simulink model "IEEE13_coord"  (R2024b)
settings: Solver=ode4  StartTime=0.0  StopTime=1.3  FixedStep=Ts  MaxStep=1e-4  RelTol=1e-4
InitFcn:
  | a=1; % Loading Factor
  | Ts=50e-6;
  | % phase to sequence conversion of RXB matrices
  | c=1*exp(sqrt(-1)*(120*pi/180));
  | T=[1 1 1;1 c*c c;1 c c*c];
  | Tinv=1/3*[1 1 1;1 c c*c;1 c*c c];
  | 
  | % Simulation data for the IEEE 13 Node Test Feeder model
  | mi2km = 1.60934;%  miles to km conversion
  | ft2km = 0.0003048; % feet to km conversion
  | ms2F = 1*1e-6/(2*pi*60);% microsiemens to Farads conversion
  | 
  | 
  | %% Configuration 601
  | % Series Resitance and Reactance - ohm/mile
  | R_601 = [0.3465 0.1560 0.1580;0.1560 0.3375 0.1535;0.1580 0.1535 0.3414];
  | X_601 = [1.1079 0.5017 0.4236;0.5017 1.0478 0.3849;0.4236 0.3849 1.0348];
  | % charging susceptance - microsiemens/mile
  | B_601 = [6.2998 -1.9958 -1.2595;-1.9958 5.9597 -0.7417;-1.2595 -0.7417 5.6386];
  | 
  | R_601 = R_601/mi2km;
  | Rseq=Tinv*R_601*T;
  | R1_601=Rseq(2,2);R0_601=Rseq(1,1);
  | 
  | L_601 = (X_601/(2*pi*60))/mi2km;
  | Lseq=Tinv*L_601*T;
  | L1_601=Lseq(2,2);L0_601=Lseq(1,1);
  | 
  | C_601 =(B_601*ms2F)/mi2km;
  | Cseq=Tinv*C_601*T;
  | C1_601=Cseq(2,2);C0_601=Cseq(1,1);
  | 
  | %% Configuration 602 - series reactance - ohm/mile
  | R_602 = [0.7526 0.1580 0.1560;0.1580 0.7475 0.1535;0.1560 0.1535 0.7436];
  | X_602 = [1.1814 0.4236 0.5017;0.4236 1.1983 0.3849;0.5017 0.3849 1.2112];
  | % charging susceptance - microsiemens/mile
  | B_602 = [5.6990 -1.0817 -1.6905;-1.0817 5.1795 -0.6588;-1.6905 -0.6588 5.4246];
  | 
  | R_602 = R_602/mi2km;
  | Rseq=Tinv*R_602*T;
  | R1_602=Rseq(2,2);R0_602=Rseq(1,1);
  | 
  | L_602 = (X_602/(2*pi*60))/mi2km;
  | Lseq=Tinv*L_602*T;
  | L1_602=Lseq(2,2);L0_602=Lseq(1,1);
  | 
  | C_602 =(B_602*ms2F)/mi2km;
  | Cseq=Tinv*C_602*T;
  | C1_602=Cseq(2,2);C0_602=Cseq(1,1);
  | %% Configuration 603 - series reactance - ohm/mile
  | R_603 = [0 0 0;0 1.3294 0.2066;0 0.2066 1.3238];
  | X_603 = [0 0 0;0 1.3471 0.4591;0 0.4591 1.3569];
  | % charging susceptance - microsiemens/mile
  | B_603 = [0 0 0;0 4.7097 -0.8999;0 -0.8999 4.6658];
  | 
  | % convert for SPS
  | R_603 = R_603/mi2km;
  | Rseq=Tinv*R_603*T;
  | R1_603=Rseq(2,2);R0_603=Rseq(1,1);
  | 
  | ... (+71 lines)
undefined symbols (not defined in the file): find_system
libraries: spsGroundLib x48, spsSeriesRLCBranchLib x46, spsThreePhaseVIMeasurementLib x19, spsControlledVoltageSourceLib x15, spsThreePhaseSeriesRLCLoadLib x7, spsVoltageMeasurementLib x6, spsOnDelayLib x6, spsThreePhasePISectionLineLib x5, spsSeriesRLCLoadLib x5, spsThreePhaseBreakerLib x5, spsMutualInductanceLib x4, spsThreePhaseSeriesRLCBranchLib x4
(part 2 of 3)

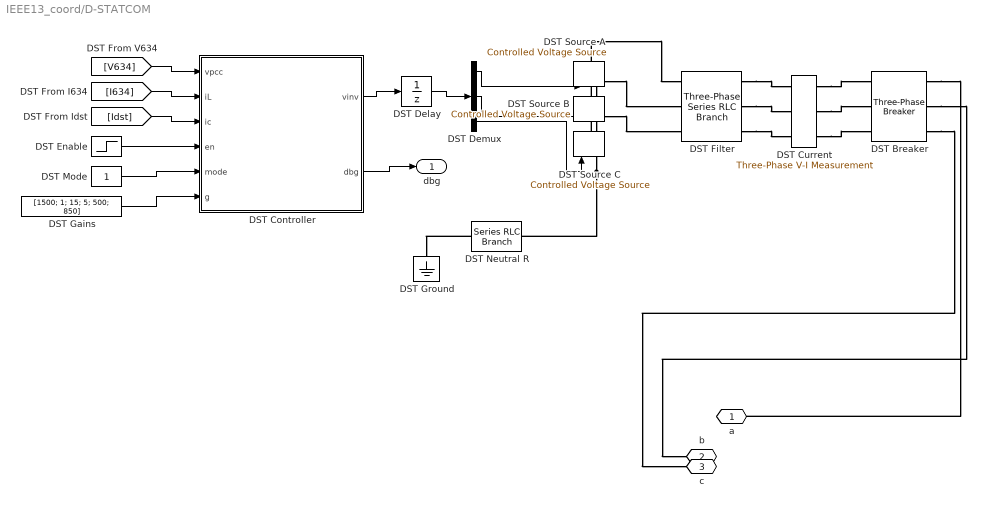
== system IEEE13_coord/D-STATCOM ==
  DST Breaker : spsThreePhaseBreakerLib/Three-Phase Breaker  InitialState=open  SwitchA=on  SwitchB=on  SwitchC=on  SwitchTimes=[100]  External=off  BreakerResistance=0.01  SnubberResistance=1e6  SnubberCapacitance=inf  Measurements=None
  DST Controller : MATLAB Function  TreatAsAtomicUnit=on
  DST Current : spsThreePhaseVIMeasurementLib/Three-Phase V-I Measurement  VoltageMeasurement=no  SetLabelV=off  LabelV=Vabc  Vpu=off  VpuLL=off  CurrentMeasurement=yes  SetLabelI=on  LabelI=Idst  Ipu=off  Pbase=100e6  Vbase=500e3  OutputType=Complex  PhasorSimulation=off  PSBequivalent=0
  DST Delay : UnitDelay  SampleTime=-1  HasFrameUpgradeWarning=on
  DST Demux : Demux  Outputs=3
  DST Enable : Step  Time=100  SampleTime=50e-6
  DST Filter : spsThreePhaseSeriesRLCBranchLib/Three-Phase Series RLC Branch  LConnTagsString=A|B|C  RConnTagsString=A|B|C  BranchType=RL  Resistance=5e-3  Inductance=0.2e-3  Capacitance=1e-6  Measurements=None
  DST Gains : Constant  Value=[1500; 1; 15; 5; 500; 850]  SampleTime=50e-6
  DST Ground : spsGroundLib/Ground  LConnTagsString=a
  DST Mode : Constant  SampleTime=50e-6
  DST Neutral R : spsSeriesRLCBranchLib/Series RLC Branch  LConnTagsString=__new0  RConnTagsString=__new0  BranchType=R  Resistance=1e6  Inductance=1e-3  SetiL0=off  InitialCurrent=0  Capacitance=1e-6  Setx0=off  InitialVoltage=0  Measurements=None
  DST Source A : spsControlledVoltageSourceLib/Controlled Voltage Source  Initialize=off  Source_Type=AC  Amplitude=0  Phase=0  Frequency=0  Measurements=None
  DST Source B : spsControlledVoltageSourceLib/Controlled Voltage Source  Initialize=off  Source_Type=AC  Amplitude=0  Phase=0  Frequency=0  Measurements=None
  DST Source C : spsControlledVoltageSourceLib/Controlled Voltage Source  Initialize=off  Source_Type=AC  Amplitude=0  Phase=0  Frequency=0  Measurements=None
  a : PMIOPort  Side=Right
  b : PMIOPort  Port=2  Side=Right
  c : PMIOPort  Port=3  Side=Right
  dbg : Outport
  wires:
  DST Mode/1 -> DST Controller/5(mode)
  DST Demux/3 -> DST Source C/1
  [V634] -> DST Controller/1(vpcc)
  [I634] -> DST Controller/2(iL)
  DST Delay/1 -> DST Demux/1
  [Idst] -> DST Controller/3(ic)
  DST Controller/1(vinv) -> DST Delay/1
  DST Gains/1 -> DST Controller/6(g)
  DST Controller/2(dbg) -> dbg/1
  DST Demux/1 -> DST Source A/1
  DST Demux/2 -> DST Source B/1
  DST Enable/1 -> DST Controller/4(en)
  connections:
  DST Breaker/RConn3 -- c/RConn1
  DST Current/RConn2 -- DST Breaker/LConn2
  DST Source B/RConn1 -- DST Filter/LConn2
  DST Source A/LConn1 -- DST Neutral R/RConn1 -- DST Source C/LConn1 -- DST Source B/LConn1
  DST Filter/RConn1 -- DST Current/LConn1
  DST Current/RConn3 -- DST Breaker/LConn3
  DST Filter/RConn3 -- DST Current/LConn3
  DST Neutral R/LConn1 -- DST Ground/LConn1
  DST Source C/RConn1 -- DST Filter/LConn3
  DST Current/RConn1 -- DST Breaker/LConn1
  DST Filter/RConn2 -- DST Current/LConn2
  DST Breaker/RConn1 -- a/RConn1
  DST Source A/RConn1 -- DST Filter/LConn1
  DST Breaker/RConn2 -- b/RConn1

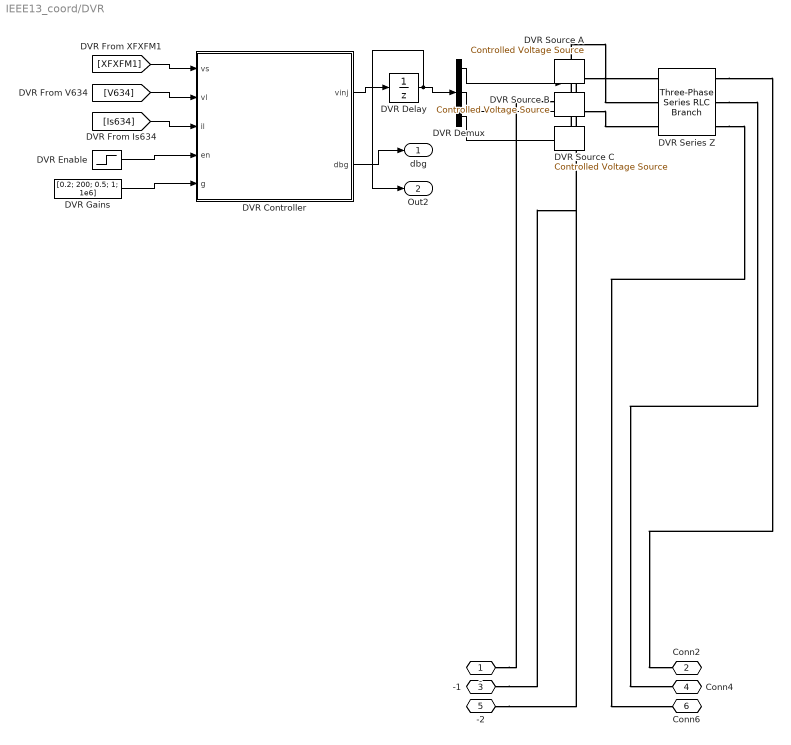
== system IEEE13_coord/DVR ==
  DVR Controller : MATLAB Function  TreatAsAtomicUnit=on
  DVR Delay : UnitDelay  SampleTime=-1  HasFrameUpgradeWarning=on
  DVR Demux : Demux  Outputs=3
  DVR Enable : Step  Time=100  SampleTime=50e-6
  DVR Gains : Constant  Value=[0.2; 200; 0.5; 1; 1e6]  SampleTime=50e-6
  DVR Series Z : spsThreePhaseSeriesRLCBranchLib/Three-Phase Series RLC Branch  LConnTagsString=A|B|C  RConnTagsString=A|B|C  BranchType=RL  Resistance=2e-3  Inductance=60e-6  Capacitance=1e-6  Measurements=None
  DVR Source A : spsControlledVoltageSourceLib/Controlled Voltage Source  Initialize=off  Source_Type=AC  Amplitude=0  Phase=0  Frequency=0  Measurements=None
  DVR Source B : spsControlledVoltageSourceLib/Controlled Voltage Source  Initialize=off  Source_Type=AC  Amplitude=0  Phase=0  Frequency=0  Measurements=None
  DVR Source C : spsControlledVoltageSourceLib/Controlled Voltage Source  Initialize=off  Source_Type=AC  Amplitude=0  Phase=0  Frequency=0  Measurements=None
  - : PMIOPort  Side=Left
  Conn2 : PMIOPort  Port=2  Side=Right
  -1 : PMIOPort  Port=3  Side=Left
  Conn4 : PMIOPort  Port=4  Side=Right
  -2 : PMIOPort  Port=5  Side=Left
  Conn6 : PMIOPort  Port=6  Side=Right
  dbg : Outport
  Out2 : Outport  Port=2
  wires:
  DVR Demux/2 -> DVR Source B/1
  [XFXFM1] -> DVR Controller/1(vs)
  DVR Gains/1 -> DVR Controller/5(g)
  [Is634] -> DVR Controller/3(il)
  DVR Delay/1 -> Out2/1, DVR Demux/1
  [V634] -> DVR Controller/2(vl)
  DVR Controller/1(vinj) -> DVR Delay/1
  DVR Enable/1 -> DVR Controller/4(en)
  DVR Demux/1 -> DVR Source A/1
  DVR Demux/3 -> DVR Source C/1
  DVR Controller/2(dbg) -> dbg/1
  connections:
  DVR Source B/RConn1 -- DVR Series Z/LConn2
  DVR Source A/RConn1 -- DVR Series Z/LConn1
  DVR Source C/RConn1 -- DVR Series Z/LConn3
  -1/RConn1 -- DVR Source B/LConn1
  -2/RConn1 -- DVR Source C/LConn1
  -/RConn1 -- DVR Source A/LConn1
  DVR Series Z/RConn2 -- Conn4/RConn1
  DVR Series Z/RConn1 -- Conn2/RConn1
  DVR Series Z/RConn3 -- Conn6/RConn1

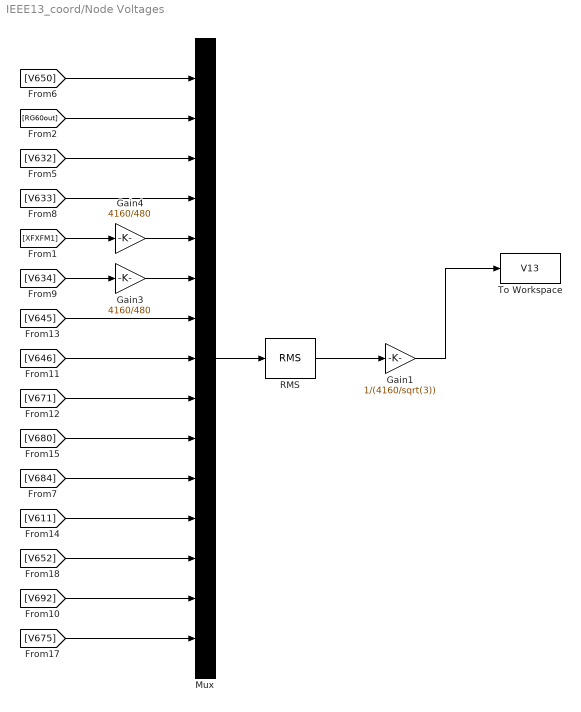
== system IEEE13_coord/Node Voltages ==
  Gain1 : Gain  Gain=1/(4160/sqrt(3))
  Gain3 : Gain  Gain=4160/480
  Gain4 : Gain  Gain=4160/480
  Mux : Mux  Inputs=15
  RMS : spsRMSLib/RMS  TrueRMS=on  Freq=60  RMSInit=120  Ts=0
  To Workspace : ToWorkspace  VariableName=V13  SampleTime=.1
  wires:
  RMS/1 -> Gain1/1
  Gain1/1 -> To Workspace/1
  Mux/1 -> RMS/1
  [V634] -> Gain3/1
  [V684] -> Mux/11
  [V675] -> Mux/15
  [V646] -> Mux/8
  [V633] -> Mux/4
  Gain3/1 -> Mux/6
  [XFXFM1] -> Gain4/1
  [V611] -> Mux/12
  [V632] -> Mux/3
  [V671] -> Mux/9
  [V680] -> Mux/10
  [V650] -> Mux/1
  [V652] -> Mux/13
  [RG60out] -> Mux/2
  [V692] -> Mux/14
  [V645] -> Mux/7
  Gain4/1 -> Mux/5

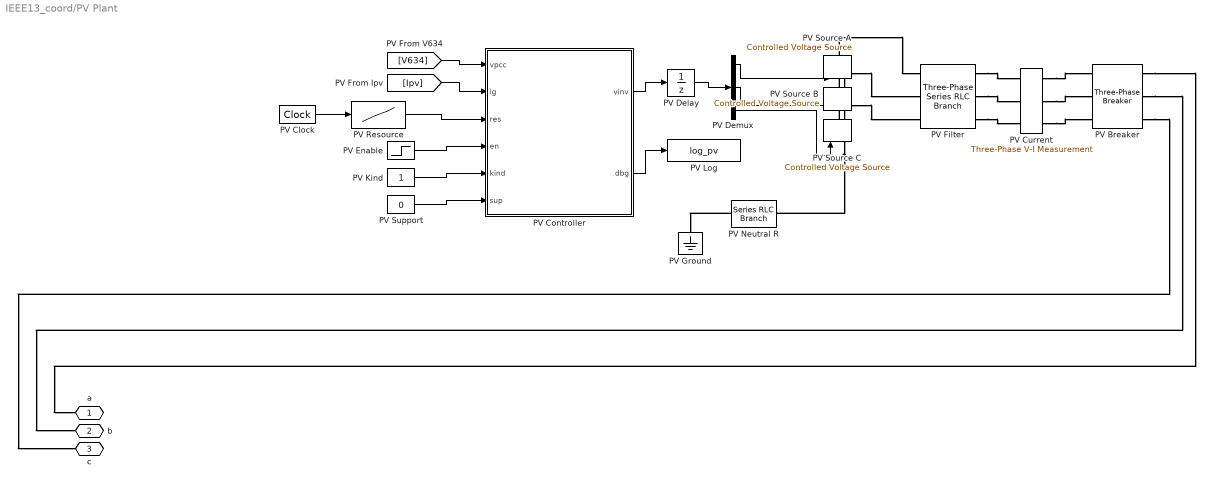
== system IEEE13_coord/PV Plant ==
  PV Breaker : spsThreePhaseBreakerLib/Three-Phase Breaker  InitialState=open  SwitchA=on  SwitchB=on  SwitchC=on  SwitchTimes=[0.2]  External=off  BreakerResistance=0.01  SnubberResistance=1e6  SnubberCapacitance=inf  Measurements=None
  PV Clock : DigitalClock  SampleTime=50e-6
  PV Controller : MATLAB Function  TreatAsAtomicUnit=on
  PV Current : spsThreePhaseVIMeasurementLib/Three-Phase V-I Measurement  VoltageMeasurement=no  SetLabelV=off  LabelV=Vabc  Vpu=off  VpuLL=off  CurrentMeasurement=yes  SetLabelI=on  LabelI=Ipv  Ipu=off  Pbase=100e6  Vbase=500e3  OutputType=Complex  PhasorSimulation=off  PSBequivalent=0
  PV Delay : UnitDelay  SampleTime=-1  HasFrameUpgradeWarning=on
  PV Demux : Demux  Outputs=3
  PV Enable : Step  Time=0.2  SampleTime=50e-6
  PV Filter : spsThreePhaseSeriesRLCBranchLib/Three-Phase Series RLC Branch  LConnTagsString=A|B|C  RConnTagsString=A|B|C  BranchType=RL  Resistance=0.01*480^2/450e3  Inductance=0.1*480^2/450e3/(2*pi*60)  Capacitance=1e-6  Measurements=None
  PV Ground : spsGroundLib/Ground  LConnTagsString=a
  PV Kind : Constant  SampleTime=50e-6
  PV Log : ToWorkspace  VariableName=log_pv  SaveFormat=Timeseries  SampleTime=-1
  PV Neutral R : spsSeriesRLCBranchLib/Series RLC Branch  LConnTagsString=__new0  RConnTagsString=__new0  BranchType=R  Resistance=1e6  Inductance=1e-3  SetiL0=off  InitialCurrent=0  Capacitance=1e-6  Setx0=off  InitialVoltage=0  Measurements=None
  PV Resource : Lookup_n-D  NumberOfTableDimensions=1  BreakpointsForDimension1=[0 100]  Table=[1000 1000]  ExtrapMethod=Clip  InternalRulePriority=Speed  RndMeth=Simplest
  PV Source A : spsControlledVoltageSourceLib/Controlled Voltage Source  Initialize=off  Source_Type=AC  Amplitude=0  Phase=0  Frequency=0  Measurements=None
  PV Source B : spsControlledVoltageSourceLib/Controlled Voltage Source  Initialize=off  Source_Type=AC  Amplitude=0  Phase=0  Frequency=0  Measurements=None
  PV Source C : spsControlledVoltageSourceLib/Controlled Voltage Source  Initialize=off  Source_Type=AC  Amplitude=0  Phase=0  Frequency=0  Measurements=None
  PV Support : Constant  Value=0  SampleTime=50e-6
  a : PMIOPort  Side=Right
  b : PMIOPort  Port=2  Side=Right
  c : PMIOPort  Port=3  Side=Right
  wires:
  PV Clock/1 -> PV Resource/1
  PV Delay/1 -> PV Demux/1
  PV Controller/2(dbg) -> PV Log/1
  [Ipv] -> PV Controller/2(ig)
  PV Enable/1 -> PV Controller/4(en)
  PV Demux/3 -> PV Source C/1
  [V634] -> PV Controller/1(vpcc)
  PV Demux/1 -> PV Source A/1
  PV Controller/1(vinv) -> PV Delay/1
  PV Demux/2 -> PV Source B/1
  PV Resource/1 -> PV Controller/3(res)
  PV Support/1 -> PV Controller/6(sup)
  PV Kind/1 -> PV Controller/5(kind)
  connections:
  PV Source A/LConn1 -- PV Neutral R/RConn1 -- PV Source C/LConn1 -- PV Source B/LConn1
  PV Current/RConn1 -- PV Breaker/LConn1
  PV Breaker/RConn1 -- a/RConn1
  PV Source B/RConn1 -- PV Filter/LConn2
  PV Filter/RConn1 -- PV Current/LConn1
  PV Source C/RConn1 -- PV Filter/LConn3
  PV Source A/RConn1 -- PV Filter/LConn1
  PV Filter/RConn3 -- PV Current/LConn3
  PV Filter/RConn2 -- PV Current/LConn2
  PV Breaker/RConn2 -- b/RConn1
  PV Neutral R/LConn1 -- PV Ground/LConn1
  PV Current/RConn2 -- PV Breaker/LConn2
  PV Current/RConn3 -- PV Breaker/LConn3
  PV Breaker/RConn3 -- c/RConn1

== system IEEE13_coord/Regulator 1 ==
  Mux : Mux  Inputs=3
  Single Phase SVR_A : Subsystem  LoadFcn=find_system(gcs,'FollowLinks', 'on', 'LookUnderMasks', 'all');  mask(Single-Phase OLTC){pNom=5e6/3, fNom=60, vNom=4160/sqrt(3), ctRatio=700, ptRatio=20, DeltaU=0.00625, TapMinMax=[-16 16], InitialTap=-10, TapSelectionTime=0.2, RegulatorOn=on, Regulator=[122/120  2/120  0.2], Comp=[3 9]}
      mask prompts: pNom "Nominal Power (VA)"; fNom "Nominal Frequency (Hz)"; vNom "Nominal Voltage (Vrms)"; ctRatio "Primary CT Rating (A)"; ptRatio "PT Ratio"; DeltaU "Voltage Step Per Tap (pu)"; TapMinMax "Minimum and Maximum Tap Positions"; InitialTap "Initial Tap Position"; TapSelectionTime "Tap Selection Time (s)"; RegulatorOn "Voltage Regulator"; Regulator "Voltage Regulator [ Vref(pu) DeadBand(pu)  Delay(s)]"; Comp "Compensator Settings [R (V) X(V)]"
      mask help:
      | Models a single-phase On Load Tap Changer (OLTC). The single-phase primary of multi-tap winding is modeled with a Variable-Ratio Transformer block.
      |
      | The transformer voltage ratio U2/U1 (in pu) is given by:
      |                 U2/U1= 1/ (1+TapPosition*DeltaU)
      | Tap position 0 corresponds to nominal voltage ratio.
      |
      | When Voltage regulator is 'on',  voltage regulator asks for a tap change if:
      |                  abs(Vm-Vref)>DeadBand/2  during a time  t > Delay.
      |
      | where 'Vm' is voltage measured at regulating point and Vref is reference voltage.
      | With line drop compensation, Vm=Vsec-Isec(R+jX)
      mask init:
      | RegulatorVref=Regulator(1);
      | RegulatorDeadBand=Regulator(2);
      | RegulatorDelay=Regulator(3);
      | Rc=Comp(1);
      | Xc=Comp(2);
      mask TypeOptions RegulatorOn: off | on
      mask Callback RegulatorOn:
      | tempMaskVis=get_param(gcb,'MaskVisibilities');
      | if strcmp(get_param(gcb,'RegulatorOn'),'on')
      | 	tempMaskVis{11}='on';
      | 	set_param(gcb,'MaskVisibilities',tempMaskVis);
      | else
      | 	tempMaskVis{11}='off';
      | 	set_param(gcb,'MaskVisibilities',tempMaskVis);
      | end
      | if strcmp(get_param(gcb,'RegulatorOn'),'on')
      | 	tempMaskVis{12}='on';
      | 	set_param(gcb,'MaskVisibilities',tempMaskVis);
      | else
      | 	tempMaskVis{12}='off';
      | 	set_param(gcb,'MaskVisibilities',tempMaskVis);
      | end
      mask DialogControl Container8 Prompt: Setup
      mask DialogControl Container13 Prompt: Regulator Parameters
      mask Display:
      | color('blue');
      | r=50;x=40;y=80;
      | th = 0:pi/100:2*pi;
      | f = r * exp(j*th) + x+j*y;
      | plot(real(f), imag(f));
      | color('red');
      | plot([-10 90],[30,130])
      | plot([75 90],[125,130])
      | plot([85 90],[115,130])
      | color('black')
      | port_label('Lconn',1,'S');port_label('Rconn',1,'L');
  Single Phase SVR_B : Subsystem  LoadFcn=find_system(gcs,'FollowLinks', 'on', 'LookUnderMasks', 'all');  mask(Single-Phase OLTC){pNom=5e6/3, fNom=60, vNom=4160/sqrt(3), ctRatio=700, ptRatio=20, DeltaU=0.00625, TapMinMax=[-16 16], InitialTap=-8, TapSelectionTime=0.2, RegulatorOn=on, Regulator=[122/120  2/120  0.2], Comp=[3 9]}
      mask prompts: pNom "Nominal Power (VA)"; fNom "Nominal Frequency (Hz)"; vNom "Nominal Voltage (Vrms)"; ctRatio "Primary CT Rating (A)"; ptRatio "PT Ratio"; DeltaU "Voltage Step Per Tap (pu)"; TapMinMax "Minimum and Maximum Tap Positions"; InitialTap "Initial Tap Position"; TapSelectionTime "Tap Selection Time (s)"; RegulatorOn "Voltage Regulator"; Regulator "Voltage Regulator [ Vref(pu) DeadBand(pu)  Delay(s)]"; Comp "Compensator Settings [R (V) X(V)]"
      mask help:
      | Models a single-phase On Load Tap Changer (OLTC). The single-phase primary of multi-tap winding is modeled with a Variable-Ratio Transformer block.
      |
      | The transformer voltage ratio U2/U1 (in pu) is given by:
      |                 U2/U1= 1/ (1+TapPosition*DeltaU)
      | Tap position 0 corresponds to nominal voltage ratio.
      |
      | When Voltage regulator is 'on',  voltage regulator asks for a tap change if:
      |                  abs(Vm-Vref)>DeadBand/2  during a time  t > Delay.
      |
      | where 'Vm' is voltage measured at regulating point and Vref is reference voltage.
      | With line drop compensation, Vm=Vsec-Isec(R+jX)
      mask init:
      | RegulatorVref=Regulator(1);
      | RegulatorDeadBand=Regulator(2);
      | RegulatorDelay=Regulator(3);
      | Rc=Comp(1);
      | Xc=Comp(2);
      mask TypeOptions RegulatorOn: off | on
      mask Callback RegulatorOn:
      | tempMaskVis=get_param(gcb,'MaskVisibilities');
      | if strcmp(get_param(gcb,'RegulatorOn'),'on')
      | 	tempMaskVis{11}='on';
      | 	set_param(gcb,'MaskVisibilities',tempMaskVis);
      | else
      | 	tempMaskVis{11}='off';
      | 	set_param(gcb,'MaskVisibilities',tempMaskVis);
      | end
      | if strcmp(get_param(gcb,'RegulatorOn'),'on')
      | 	tempMaskVis{12}='on';
      | 	set_param(gcb,'MaskVisibilities',tempMaskVis);
      | else
      | 	tempMaskVis{12}='off';
      | 	set_param(gcb,'MaskVisibilities',tempMaskVis);
      | end
      mask DialogControl Container8 Prompt: Setup
      mask DialogControl Container13 Prompt: Regulator Parameters
      mask Display:
      | color('blue');
      | r=50;x=40;y=80;
      | th = 0:pi/100:2*pi;
      | f = r * exp(j*th) + x+j*y;
      | plot(real(f), imag(f));
      | color('red');
      | plot([-10 90],[30,130])
      | plot([75 90],[125,130])
      | plot([85 90],[115,130])
      | color('black')
      | port_label('Lconn',1,'S');port_label('Rconn',1,'L');
  Single Phase SVR_C : Subsystem  LoadFcn=find_system(gcs,'FollowLinks', 'on', 'LookUnderMasks', 'all');  mask(Single-Phase OLTC){pNom=5e6/3, fNom=60, vNom=4160/sqrt(3), ctRatio=700, ptRatio=20, DeltaU=0.00625, TapMinMax=[-16 16], InitialTap=-11, TapSelectionTime=0.2, RegulatorOn=on, Regulator=[122/120  2/120  0.2], Comp=[3 9]}
      mask prompts: pNom "Nominal Power (VA)"; fNom "Nominal Frequency (Hz)"; vNom "Nominal Voltage (Vrms)"; ctRatio "Primary CT Rating (A)"; ptRatio "PT Ratio"; DeltaU "Voltage Step Per Tap (pu)"; TapMinMax "Minimum and Maximum Tap Positions"; InitialTap "Initial Tap Position"; TapSelectionTime "Tap Selection Time (s)"; RegulatorOn "Voltage Regulator"; Regulator "Voltage Regulator [ Vref(pu) DeadBand(pu)  Delay(s)]"; Comp "Compensator Settings [R (V) X(V)]"
      mask help:
      | Models a single-phase On Load Tap Changer (OLTC). The single-phase primary of multi-tap winding is modeled with a Variable-Ratio Transformer block.
      |
      | The transformer voltage ratio U2/U1 (in pu) is given by:
      |                 U2/U1= 1/ (1+TapPosition*DeltaU)
      | Tap position 0 corresponds to nominal voltage ratio.
      |
      | When Voltage regulator is 'on',  voltage regulator asks for a tap change if:
      |                  abs(Vm-Vref)>DeadBand/2  during a time  t > Delay.
      |
      | where 'Vm' is voltage measured at regulating point and Vref is reference voltage.
      | With line drop compensation, Vm=Vsec-Isec(R+jX)
      mask init:
      | RegulatorVref=Regulator(1);
      | RegulatorDeadBand=Regulator(2);
      | RegulatorDelay=Regulator(3);
      | Rc=Comp(1);
      | Xc=Comp(2);
      mask TypeOptions RegulatorOn: off | on
      mask Callback RegulatorOn:
      | tempMaskVis=get_param(gcb,'MaskVisibilities');
      | if strcmp(get_param(gcb,'RegulatorOn'),'on')
      | 	tempMaskVis{11}='on';
      | 	set_param(gcb,'MaskVisibilities',tempMaskVis);
      | else
      | 	tempMaskVis{11}='off';
      | 	set_param(gcb,'MaskVisibilities',tempMaskVis);
      | end
      | if strcmp(get_param(gcb,'RegulatorOn'),'on')
      | 	tempMaskVis{12}='on';
      | 	set_param(gcb,'MaskVisibilities',tempMaskVis);
      | else
      | 	tempMaskVis{12}='off';
      | 	set_param(gcb,'MaskVisibilities',tempMaskVis);
      | end
      mask DialogControl Container8 Prompt: Setup
      mask DialogControl Container13 Prompt: Regulator Parameters
      mask Display:
      | color('blue');
      | r=50;x=40;y=80;
      | th = 0:pi/100:2*pi;
      | f = r * exp(j*th) + x+j*y;
      | plot(real(f), imag(f));
      | color('red');
      | plot([-10 90],[30,130])
      | plot([75 90],[125,130])
      | plot([85 90],[115,130])
      | color('black')
      | port_label('Lconn',1,'S');port_label('Rconn',1,'L');
  A : PMIOPort  Side=Left
  a : PMIOPort  Port=2  Side=Right
  B : PMIOPort  Port=3  Side=Left
  b : PMIOPort  Port=4  Side=Right
  C : PMIOPort  Port=5  Side=Left
  c : PMIOPort  Port=6  Side=Right
  Tap : Outport
  wires:
  Mux/1 -> Tap/1
  Single Phase SVR_C/1(Tap) -> Mux/3
  Single Phase SVR_B/1(Tap) -> Mux/2
  Single Phase SVR_A/1(Tap) -> Mux/1
  connections:
  Single Phase SVR_C/RConn1 -- c/RConn1
  Single Phase SVR_C/LConn1 -- C/RConn1
  Single Phase SVR_B/RConn1 -- b/RConn1
  Single Phase SVR_B/LConn1 -- B/RConn1
  Single Phase SVR_A/LConn1 -- A/RConn1
  Single Phase SVR_A/RConn1 -- a/RConn1

== system IEEE13_coord/Regulator Taps  ==
  note: Here the taps of the Voltage Regulator are on primary side of transformers unlike in Benchmark document where taps are considered on secondary of transformer. Therefore the values used are negative of what is used in Benchmark document. Also the direction of Tap Operation will be in opposite direction as compared to Regulator having taps on secondary side of transformer.
  Band Width : Constant  Value=2
  Band Width1 : Constant  Value=2
  Gain : Gain  Gain=1/2
  Gain2 : Gain  Gain=1/2
  Scope3 : Scope  NumInputPorts=5
  Sum : Sum  Inputs=|++
  Sum1 : Sum  Inputs=|+-
  Tap : Scope
  Vref : Constant  Value=122
  Vref1 : Constant  Value=122
  wires:
  [Rg1] -> Tap/1
  Vref/1 -> Sum/1
  Band Width/1 -> Gain/1
  Gain/1 -> Sum/2
  Gain2/1 -> Sum1/2
  Band Width1/1 -> Gain2/1
  Vref1/1 -> Sum1/1
  Sum/1 -> Scope3/1  "Upper Limit"
  [Vr1a] -> Scope3/2  "Vra"
  [Vr1b] -> Scope3/3  "Vrb"
  [Vr1c] -> Scope3/4  "Vrc"
  Sum1/1 -> Scope3/5  "Lower Limit"

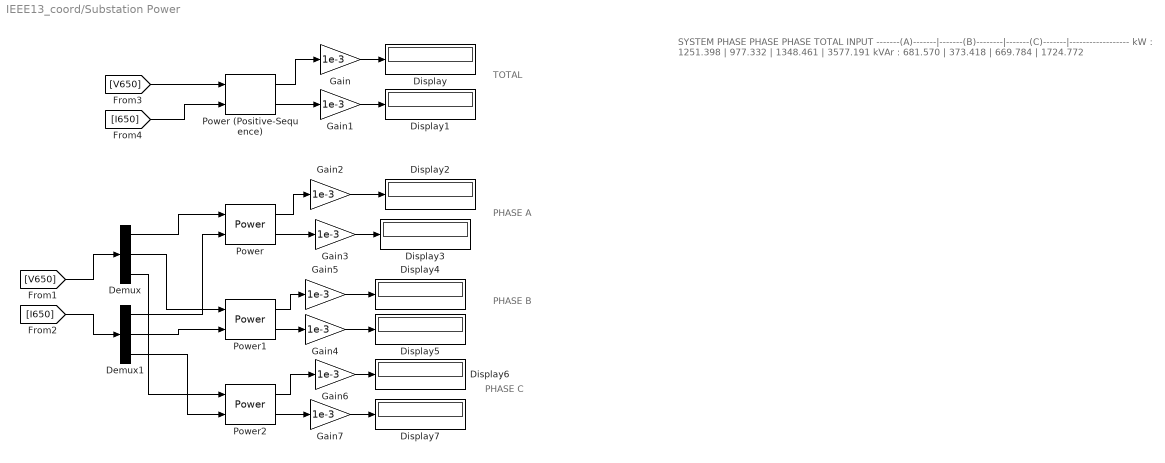
== system IEEE13_coord/Substation Power ==
  note: SYSTEM PHASE PHASE PHASE TOTAL
      | INPUT -------(A)-------|-------(B)--------|-------(C)-------|------------------
      | kW : 1251.398 | 977.332 | 1348.461 | 3577.191
      | kVAr : 681.570 | 373.418 | 669.784 | 1724.772
  note: PHASE A
  note: PHASE C
  note: PHASE B
  note: TOTAL
  Demux : Demux  Outputs=3
  Demux1 : Demux  Outputs=3
  Display{,1..7} (8 alike) : Display
  Gain{,1..7} (8 alike) : Gain  Gain=1e-3
  Power : spsPowerLib/Power  Freq=60  Vinit=[1, 0]  Iinit=[1, 0]  Ts=0
  Power (Positive-Sequence) : spsPowerPositiveSequenceLib/Power (Positive-Sequence)  Freq=60  Vinit=[0, 0]  Iinit=[0, 0]  Ts=Ts
      settings: LibrarySourceBlock=|
      | sps_lib/Sensors and Measurements/Power
      | (Positive-Sequence)
  Power1 : spsPowerLib/Power  Freq=60  Vinit=[1, 0]  Iinit=[1, 0]  Ts=0
  Power2 : spsPowerLib/Power  Freq=60  Vinit=[1, 0]  Iinit=[1, 0]  Ts=0
  wires:
  [I650] -> Power (Positive-Sequence)/2
  [V650] -> Power (Positive-Sequence)/1
  Power (Positive-Sequence)/1 -> Gain/1
  Power (Positive-Sequence)/2 -> Gain1/1
  [V650] -> Demux/1
  [I650] -> Demux1/1
  Demux/1 -> Power/1
  Demux1/1 -> Power/2
  Demux/2 -> Power1/1
  Demux1/2 -> Power1/2
  Demux/3 -> Power2/1
  Demux1/3 -> Power2/2
  Power/1 -> Gain2/1
  Power/2 -> Gain3/1
  Power1/1 -> Gain5/1
  Power1/2 -> Gain4/1
  Power2/1 -> Gain6/1
  Power2/2 -> Gain7/1
  Gain/1 -> Display/1
  Gain1/1 -> Display1/1
  Gain2/1 -> Display2/1
  Gain3/1 -> Display3/1
  Gain4/1 -> Display5/1
  Gain5/1 -> Display4/1
  Gain6/1 -> Display6/1
  Gain7/1 -> Display7/1

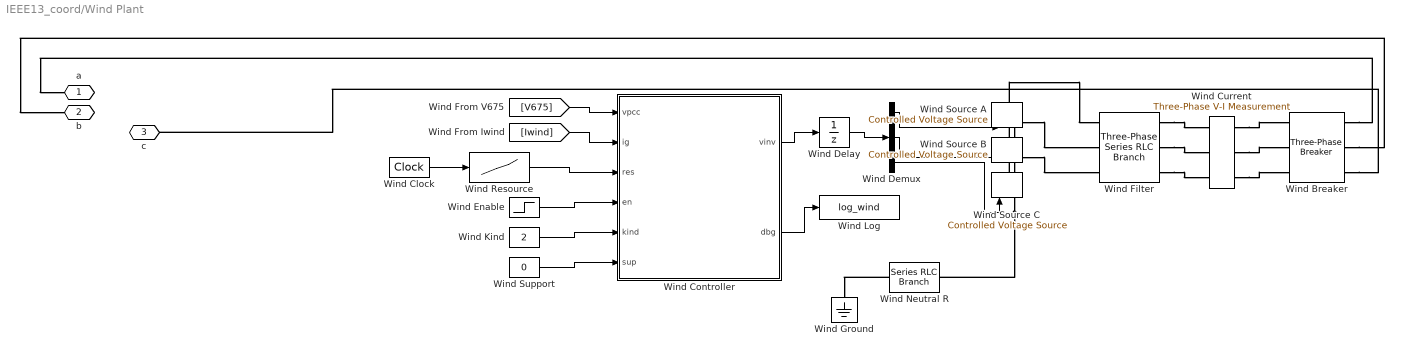
== system IEEE13_coord/Wind Plant ==
  Wind Breaker : spsThreePhaseBreakerLib/Three-Phase Breaker  InitialState=open  SwitchA=on  SwitchB=on  SwitchC=on  SwitchTimes=[0.2]  External=off  BreakerResistance=0.01  SnubberResistance=1e6  SnubberCapacitance=inf  Measurements=None
  Wind Clock : DigitalClock  SampleTime=50e-6
  Wind Controller : MATLAB Function  TreatAsAtomicUnit=on
  Wind Current : spsThreePhaseVIMeasurementLib/Three-Phase V-I Measurement  VoltageMeasurement=no  SetLabelV=off  LabelV=Vabc  Vpu=off  VpuLL=off  CurrentMeasurement=yes  SetLabelI=on  LabelI=Iwind  Ipu=off  Pbase=100e6  Vbase=500e3  OutputType=Complex  PhasorSimulation=off  PSBequivalent=0
  Wind Delay : UnitDelay  SampleTime=-1  HasFrameUpgradeWarning=on
  Wind Demux : Demux  Outputs=3
  Wind Enable : Step  Time=0.2  SampleTime=50e-6
  Wind Filter : spsThreePhaseSeriesRLCBranchLib/Three-Phase Series RLC Branch  LConnTagsString=A|B|C  RConnTagsString=A|B|C  BranchType=RL  Resistance=0.01*4160^2/550e3  Inductance=0.1*4160^2/550e3/(2*pi*60)  Capacitance=1e-6  Measurements=None
  Wind Ground : spsGroundLib/Ground  LConnTagsString=a
  Wind Kind : Constant  Value=2  SampleTime=50e-6
  Wind Log : ToWorkspace  VariableName=log_wind  SaveFormat=Timeseries  SampleTime=-1
  Wind Neutral R : spsSeriesRLCBranchLib/Series RLC Branch  LConnTagsString=__new0  RConnTagsString=__new0  BranchType=R  Resistance=1e6  Inductance=1e-3  SetiL0=off  InitialCurrent=0  Capacitance=1e-6  Setx0=off  InitialVoltage=0  Measurements=None
  Wind Resource : Lookup_n-D  NumberOfTableDimensions=1  BreakpointsForDimension1=[0 100]  Table=[12 12]  ExtrapMethod=Clip  InternalRulePriority=Speed  RndMeth=Simplest
  Wind Source A : spsControlledVoltageSourceLib/Controlled Voltage Source  Initialize=off  Source_Type=AC  Amplitude=0  Phase=0  Frequency=0  Measurements=None
  Wind Source B : spsControlledVoltageSourceLib/Controlled Voltage Source  Initialize=off  Source_Type=AC  Amplitude=0  Phase=0  Frequency=0  Measurements=None
  Wind Source C : spsControlledVoltageSourceLib/Controlled Voltage Source  Initialize=off  Source_Type=AC  Amplitude=0  Phase=0  Frequency=0  Measurements=None
  Wind Support : Constant  Value=0  SampleTime=50e-6
  a : PMIOPort  Side=Right
  b : PMIOPort  Port=2  Side=Right
  c : PMIOPort  Port=3  Side=Right
  wires:
  Wind Demux/1 -> Wind Source A/1
  [Iwind] -> Wind Controller/2(ig)
  Wind Controller/1(vinv) -> Wind Delay/1
  Wind Demux/3 -> Wind Source C/1
  [V675] -> Wind Controller/1(vpcc)
  Wind Delay/1 -> Wind Demux/1
  Wind Resource/1 -> Wind Controller/3(res)
  Wind Enable/1 -> Wind Controller/4(en)
  Wind Support/1 -> Wind Controller/6(sup)
  Wind Kind/1 -> Wind Controller/5(kind)
  Wind Controller/2(dbg) -> Wind Log/1
  Wind Clock/1 -> Wind Resource/1
  Wind Demux/2 -> Wind Source B/1
  connections:
  Wind Source A/LConn1 -- Wind Neutral R/RConn1 -- Wind Source C/LConn1 -- Wind Source B/LConn1
  Wind Filter/RConn3 -- Wind Current/LConn3
  Wind Current/RConn2 -- Wind Breaker/LConn2
  Wind Source B/RConn1 -- Wind Filter/LConn2
  Wind Filter/RConn2 -- Wind Current/LConn2
  Wind Breaker/RConn3 -- c/RConn1
  Wind Filter/RConn1 -- Wind Current/LConn1
  Wind Source C/RConn1 -- Wind Filter/LConn3
  Wind Current/RConn1 -- Wind Breaker/LConn1
  Wind Neutral R/LConn1 -- Wind Ground/LConn1
  Wind Source A/RConn1 -- Wind Filter/LConn1
  Wind Breaker/RConn2 -- b/RConn1
  Wind Current/RConn3 -- Wind Breaker/LConn3
  Wind Breaker/RConn1 -- a/RConn1

== system IEEE13_coord/Regulator 1/Single Phase SVR_A ==
  Line Drop Compensator : Subsystem
  Transformer with Taps : Subsystem
  Voltage Regulator Control : Subsystem
  S : PMIOPort  Tag=PMCPort  Side=Left
  L : PMIOPort  Tag=PMCPort  Port=2  Side=Right
  Tap : Outport  VectorParamsAs1DForOutWhenUnconnected=off
  tag scope: Vr1a=global
  wires:
  Line Drop Compensator/1(Vm) -> Voltage Regulator Control/1(Vm), [Vr1a]
  Voltage Regulator Control/2(Tap) -> Tap/1
  Voltage Regulator Control/1(N) -> Transformer with Taps/1(N)
  Transformer with Taps/1(Isec) -> Line Drop Compensator/1(Isec)
  Transformer with Taps/2(Vsec) -> Line Drop Compensator/2(Vsec)
  connections:
  Transformer with Taps/RConn1 -- L/RConn1
  S/RConn1 -- Transformer with Taps/LConn1

== system IEEE13_coord/Regulator 1/Single Phase SVR_B ==
  Line Drop Compensator : Subsystem
  Transformer with Taps : Subsystem
  Voltage Regulator Control : Subsystem
  S : PMIOPort  Tag=PMCPort  Side=Left
  L : PMIOPort  Tag=PMCPort  Port=2  Side=Right
  Tap : Outport  VectorParamsAs1DForOutWhenUnconnected=off
  tag scope: Vr1b=global
  wires:
  Transformer with Taps/2(Vsec) -> Line Drop Compensator/2(Vsec)
  Transformer with Taps/1(Isec) -> Line Drop Compensator/1(Isec)
  Voltage Regulator Control/1(N) -> Transformer with Taps/1(N)
  Voltage Regulator Control/2(Tap) -> Tap/1
  Line Drop Compensator/1(Vm) -> [Vr1b], Voltage Regulator Control/1(Vm)
  connections:
  S/RConn1 -- Transformer with Taps/LConn1
  Transformer with Taps/RConn1 -- L/RConn1

== system IEEE13_coord/Regulator 1/Single Phase SVR_C ==
  Line Drop Compensator : Subsystem
  Transformer with Taps : Subsystem
  Voltage Regulator Control : Subsystem
  S : PMIOPort  Tag=PMCPort  Side=Left
  L : PMIOPort  Tag=PMCPort  Port=2  Side=Right
  Tap : Outport  VectorParamsAs1DForOutWhenUnconnected=off
  tag scope: Vr1c=global
  wires:
  Line Drop Compensator/1(Vm) -> Voltage Regulator Control/1(Vm), [Vr1c]
  Voltage Regulator Control/2(Tap) -> Tap/1
  Voltage Regulator Control/1(N) -> Transformer with Taps/1(N)
  Transformer with Taps/1(Isec) -> Line Drop Compensator/1(Isec)
  Transformer with Taps/2(Vsec) -> Line Drop Compensator/2(Vsec)
  connections:
  Transformer with Taps/RConn1 -- L/RConn1
  S/RConn1 -- Transformer with Taps/LConn1

== system IEEE13_coord/Regulator 1/Single Phase SVR_A/Line Drop Compensator ==
  note: Vm=Vsec-Isec(Rc+jXc)
  Isec : Inport
  Vsec : Inport  Port=2
  "        " : spsLinearTransformerLib/Linear Transformer  UNITS=SI  NominalPower=[pNom fNom]  winding1=[vNom/ptRatio 1e-7 1e-8]  winding2=[vNom/ptRatio 1e-7 1e-8]  ThreeWindings=off  winding3=[3.15e+005 0.7938 0.084225]  RmLm=[1e5 1e5]  Measurements=None  DataType=on
  "CTS  " : spsControlledCurrentSourceLib/Controlled Current Source  Initialize=on  Source_Type=AC  Amplitude=0  Phase=0  Frequency=0  Measurements=None
  "PTS  " : spsControlledVoltageSourceLib/Controlled Voltage Source  Initialize=on  Source_Type=AC  Amplitude=0  Phase=0  Frequency=0  Measurements=None
  RMS : spsRMSLib/RMS  TrueRMS=on  Freq=60  RMSInit=120  Ts=0
  Raux : spsSeriesRLCBranchLib/Series RLC Branch  LConnTagsString=__new0  RConnTagsString=__new0  BranchType=R  Resistance=1e3  Inductance=1.6 / (120*pi)  SetiL0=off  InitialCurrent=0  Capacitance=1e-6  Setx0=off  InitialVoltage=0  Measurements=None
  Rc+jXc : spsSeriesRLCBranchLib/Series RLC Branch  LConnTagsString=__new0  RConnTagsString=__new0  BranchType=RL  Resistance=Rc  Inductance=Xc / (2*pi*fNom)  SetiL0=off  InitialCurrent=0  Capacitance=1e-6  Setx0=off  InitialVoltage=0  Measurements=None
  VRelay : spsVoltageMeasurementLib/Voltage Measurement  PhasorSimulation=off  OutputType=Complex  PSBequivalent=0
  Vm : Outport
  wires:
  RMS/1 -> Vm/1
  VRelay/1 -> RMS/1
  Isec/1 -> "CTS  "/1
  Vsec/1 -> "PTS  "/1
  connections:
  "PTS  "/RConn1 -- "        "/RConn1
  "        "/RConn2 -- VRelay/LConn1
  Raux/LConn1 -- Rc+jXc/LConn1 -- "        "/LConn1 -- "CTS  "/RConn1
  Rc+jXc/RConn1 -- Raux/RConn1 -- "CTS  "/LConn1 -- "        "/LConn2
  VRelay/LConn2 -- "PTS  "/LConn1

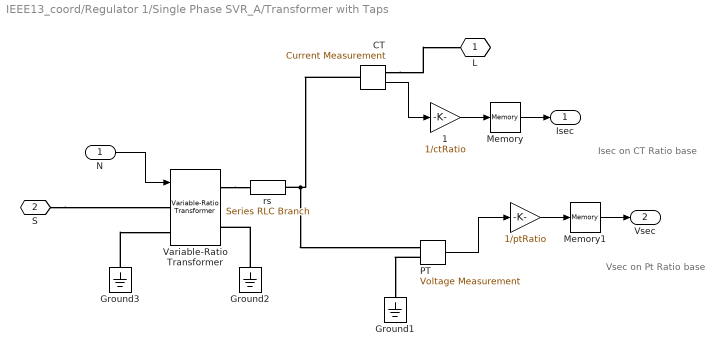
== system IEEE13_coord/Regulator 1/Single Phase SVR_A/Transformer with Taps ==
  note: Vsec on Pt Ratio base
  note: Isec on CT Ratio base
  N : Inport
  "    " : Gain  Gain=1/ptRatio
  " 1" : Gain  Gain=1/ctRatio
  CT : spsCurrentMeasurementLib/Current Measurement  PhasorSimulation=off  OutputType=Complex  PSBequivalent=0
  Ground1 : spsGroundLib/Ground  LConnTagsString=a
  Ground2 : spsGroundLib/Ground  LConnTagsString=a
  Ground3 : spsGroundLib/Ground  LConnTagsString=a
  Memory : Memory
  Memory1 : Memory
  PT : spsVoltageMeasurementLib/Voltage Measurement  PhasorSimulation=off  OutputType=Complex  PSBequivalent=0
  "Variable-Ratio Transformer " : spsVariableRatioTransformerLib/Variable-Ratio Transformer
      settings: LibrarySourceBlock=|
      | sps_lib/Passives/Variable-Ratio
      | Transformer
  rs : spsSeriesRLCBranchLib/Series RLC Branch  LConnTagsString=__new0  RConnTagsString=__new0  BranchType=R  Resistance=1e-6  Inductance=1e-3  SetiL0=off  InitialCurrent=0  Capacitance=1e-6  Setx0=off  InitialVoltage=0  Measurements=None
  L : PMIOPort  Tag=PMCPort  Side=Right
  S : PMIOPort  Port=2  Side=Left
  Isec : Outport
  Vsec : Outport  Port=2
  wires:
  "    "/1 -> Memory1/1
  PT/1 -> "    "/1
  CT/1 -> " 1"/1
  " 1"/1 -> Memory/1
  N/1 -> "Variable-Ratio Transformer "/1
  Memory1/1 -> Vsec/1
  Memory/1 -> Isec/1
  connections:
  PT/LConn2 -- Ground1/LConn1
  rs/RConn1 -- CT/LConn1 -- PT/LConn1
  CT/RConn1 -- L/RConn1
  "Variable-Ratio Transformer "/RConn1 -- rs/LConn1
  Ground3/LConn1 -- "Variable-Ratio Transformer "/LConn2
  Ground2/LConn1 -- "Variable-Ratio Transformer "/RConn2
  S/RConn1 -- "Variable-Ratio Transformer "/LConn1

== system IEEE13_coord/Regulator 1/Single Phase SVR_A/Voltage Regulator Control ==
  note: N= 1/ (1+TapPosition*DeltaU)
  Vm : Inport
  1 : Constant
  Constant : Constant  Value=RegulatorOn
  Constant5 : Constant
  Product : Product  Inputs=/*
  Sum : Sum
  Tap Changer Control : Subsystem  mask(Tap Changer Control){MinMaxTap=TapMinMax, InitialPosition=InitialTap, MecDelay=TapSelectionTime}
      mask prompts: MinMaxTap "Minimum and maximum tap number [ Min  Max ] :"; InitialPosition "Initial tap position"; MecDelay "Mechanical delay time"
      mask init:
      | if MecDelay<=0,
      | 	MecDelay=1/60;
      | end
  Voltage change per tap : Gain  Gain=DeltaU
  Voltage regulator : Subsystem  mask{Vref=RegulatorVref*120, DeadBand=RegulatorDeadBand*120, TimeDelay=RegulatorDelay}
      mask prompts: Vref "Vref (on 120v base)"; DeadBand "Deadband (on 120v base)"; TimeDelay "Time delay (s)"
  N : Outport
  Tap : Outport  Port=2
  wires:
  Vm/1 -> Voltage regulator/1(Vmes (pu))
  Product/1 -> N/1
  Constant/1 -> Voltage regulator/3(RegOn)
  Tap Changer Control/2(Ready) -> Voltage regulator/2(Ready)
  Voltage change per tap/1 -> Sum/2
  Constant5/1 -> Sum/1
  Voltage regulator/1(Up) -> Tap Changer Control/1("Up ")
  Tap Changer Control/1(TapNo) -> Voltage change per tap/1, Tap/1  "Tap"
  1/1 -> Product/2
  Sum/1 -> Product/1
  Voltage regulator/2(Down) -> Tap Changer Control/2("Down ")

== system IEEE13_coord/Regulator 1/Single Phase SVR_B/Line Drop Compensator ==
  note: Vm=Vsec-Isec(Rc+jXc)
  Isec : Inport
  Vsec : Inport  Port=2
  "        " : spsLinearTransformerLib/Linear Transformer  UNITS=SI  NominalPower=[pNom fNom]  winding1=[vNom/ptRatio 1e-7 1e-8]  winding2=[vNom/ptRatio 1e-7 1e-8]  ThreeWindings=off  winding3=[3.15e+005 0.7938 0.084225]  RmLm=[1e5 1e5]  Measurements=None  DataType=on
  "CTS  " : spsControlledCurrentSourceLib/Controlled Current Source  Initialize=on  Source_Type=AC  Amplitude=0  Phase=0  Frequency=0  Measurements=None
  "PTS  " : spsControlledVoltageSourceLib/Controlled Voltage Source  Initialize=on  Source_Type=AC  Amplitude=0  Phase=0  Frequency=0  Measurements=None
  RMS : spsRMSLib/RMS  TrueRMS=on  Freq=60  RMSInit=120  Ts=0
  Raux : spsSeriesRLCBranchLib/Series RLC Branch  LConnTagsString=__new0  RConnTagsString=__new0  BranchType=R  Resistance=1e3  Inductance=1.6 / (120*pi)  SetiL0=off  InitialCurrent=0  Capacitance=1e-6  Setx0=off  InitialVoltage=0  Measurements=None
  Rc+jXc : spsSeriesRLCBranchLib/Series RLC Branch  LConnTagsString=__new0  RConnTagsString=__new0  BranchType=RL  Resistance=Rc  Inductance=Xc / (2*pi*fNom)  SetiL0=off  InitialCurrent=0  Capacitance=1e-6  Setx0=off  InitialVoltage=0  Measurements=None
  VRelay : spsVoltageMeasurementLib/Voltage Measurement  PhasorSimulation=off  OutputType=Complex  PSBequivalent=0
  Vm : Outport
  wires:
  Vsec/1 -> "PTS  "/1
  Isec/1 -> "CTS  "/1
  VRelay/1 -> RMS/1
  RMS/1 -> Vm/1
  connections:
  VRelay/LConn2 -- "PTS  "/LConn1
  "        "/LConn2 -- "CTS  "/LConn1 -- Raux/RConn1 -- Rc+jXc/RConn1
  "CTS  "/RConn1 -- "        "/LConn1 -- Rc+jXc/LConn1 -- Raux/LConn1
  "        "/RConn2 -- VRelay/LConn1
  "PTS  "/RConn1 -- "        "/RConn1

== system IEEE13_coord/Regulator 1/Single Phase SVR_B/Transformer with Taps ==
  note: Isec on CT Ratio base
  note: Vsec on Pt Ratio base
  N : Inport
  "    " : Gain  Gain=1/ptRatio
  " 1" : Gain  Gain=1/ctRatio
  CT : spsCurrentMeasurementLib/Current Measurement  PhasorSimulation=off  OutputType=Complex  PSBequivalent=0
  Ground1 : spsGroundLib/Ground  LConnTagsString=a
  Ground2 : spsGroundLib/Ground  LConnTagsString=a
  Ground3 : spsGroundLib/Ground  LConnTagsString=a
  Memory : Memory
  Memory1 : Memory
  PT : spsVoltageMeasurementLib/Voltage Measurement  PhasorSimulation=off  OutputType=Complex  PSBequivalent=0
  "Variable-Ratio Transformer " : spsVariableRatioTransformerLib/Variable-Ratio Transformer
      settings: LibrarySourceBlock=|
      | sps_lib/Passives/Variable-Ratio
      | Transformer
  rs : spsSeriesRLCBranchLib/Series RLC Branch  LConnTagsString=__new0  RConnTagsString=__new0  BranchType=R  Resistance=1e-6  Inductance=1e-3  SetiL0=off  InitialCurrent=0  Capacitance=1e-6  Setx0=off  InitialVoltage=0  Measurements=None
  L : PMIOPort  Tag=PMCPort  Side=Right
  S : PMIOPort  Port=2  Side=Left
  Isec : Outport
  Vsec : Outport  Port=2
  wires:
  Memory/1 -> Isec/1
  Memory1/1 -> Vsec/1
  N/1 -> "Variable-Ratio Transformer "/1
  " 1"/1 -> Memory/1
  CT/1 -> " 1"/1
  PT/1 -> "    "/1
  "    "/1 -> Memory1/1
  connections:
  S/RConn1 -- "Variable-Ratio Transformer "/LConn1
  Ground2/LConn1 -- "Variable-Ratio Transformer "/RConn2
  Ground3/LConn1 -- "Variable-Ratio Transformer "/LConn2
  "Variable-Ratio Transformer "/RConn1 -- rs/LConn1
  CT/RConn1 -- L/RConn1
  PT/LConn1 -- CT/LConn1 -- rs/RConn1
  PT/LConn2 -- Ground1/LConn1

== system IEEE13_coord/Regulator 1/Single Phase SVR_B/Voltage Regulator Control ==
  note: N= 1/ (1+TapPosition*DeltaU)
  Vm : Inport
  1 : Constant
  Constant : Constant  Value=RegulatorOn
  Constant5 : Constant
  Product : Product  Inputs=/*
  Sum : Sum
  Tap Changer Control : Subsystem  mask(Tap Changer Control){MinMaxTap=TapMinMax, InitialPosition=InitialTap, MecDelay=TapSelectionTime}
      mask prompts: MinMaxTap "Minimum and maximum tap number [ Min  Max ] :"; InitialPosition "Initial tap position"; MecDelay "Mechanical delay time"
      mask init:
      | if MecDelay<=0,
      | 	MecDelay=1/60;
      | end
  Voltage change per tap : Gain  Gain=DeltaU
  Voltage regulator : Subsystem  mask{Vref=RegulatorVref*120, DeadBand=RegulatorDeadBand*120, TimeDelay=RegulatorDelay}
      mask prompts: Vref "Vref (on 120v base)"; DeadBand "Deadband (on 120v base)"; TimeDelay "Time delay (s)"
  N : Outport
  Tap : Outport  Port=2
  wires:
  Voltage regulator/2(Down) -> Tap Changer Control/2("Down ")
  Sum/1 -> Product/1
  1/1 -> Product/2
  Tap Changer Control/1(TapNo) -> Tap/1, Voltage change per tap/1  "Tap"
  Voltage regulator/1(Up) -> Tap Changer Control/1("Up ")
  Constant5/1 -> Sum/1
  Voltage change per tap/1 -> Sum/2
  Tap Changer Control/2(Ready) -> Voltage regulator/2(Ready)
  Constant/1 -> Voltage regulator/3(RegOn)
  Product/1 -> N/1
  Vm/1 -> Voltage regulator/1(Vmes (pu))

== system IEEE13_coord/Regulator 1/Single Phase SVR_C/Line Drop Compensator ==
  note: Vm=Vsec-Isec(Rc+jXc)
  Isec : Inport
  Vsec : Inport  Port=2
  "        " : spsLinearTransformerLib/Linear Transformer  UNITS=SI  NominalPower=[pNom fNom]  winding1=[vNom/ptRatio 1e-7 1e-8]  winding2=[vNom/ptRatio 1e-7 1e-8]  ThreeWindings=off  winding3=[3.15e+005 0.7938 0.084225]  RmLm=[1e5 1e5]  Measurements=None  DataType=on
  "CTS  " : spsControlledCurrentSourceLib/Controlled Current Source  Initialize=on  Source_Type=AC  Amplitude=0  Phase=0  Frequency=0  Measurements=None
  "PTS  " : spsControlledVoltageSourceLib/Controlled Voltage Source  Initialize=on  Source_Type=AC  Amplitude=0  Phase=0  Frequency=0  Measurements=None
  RMS : spsRMSLib/RMS  TrueRMS=on  Freq=60  RMSInit=120  Ts=0
  Raux : spsSeriesRLCBranchLib/Series RLC Branch  LConnTagsString=__new0  RConnTagsString=__new0  BranchType=R  Resistance=1e3  Inductance=1.6 / (120*pi)  SetiL0=off  InitialCurrent=0  Capacitance=1e-6  Setx0=off  InitialVoltage=0  Measurements=None
  Rc+jXc : spsSeriesRLCBranchLib/Series RLC Branch  LConnTagsString=__new0  RConnTagsString=__new0  BranchType=RL  Resistance=Rc  Inductance=Xc / (2*pi*fNom)  SetiL0=off  InitialCurrent=0  Capacitance=1e-6  Setx0=off  InitialVoltage=0  Measurements=None
  VRelay : spsVoltageMeasurementLib/Voltage Measurement  PhasorSimulation=off  OutputType=Complex  PSBequivalent=0
  Vm : Outport
  wires:
  RMS/1 -> Vm/1
  VRelay/1 -> RMS/1
  Isec/1 -> "CTS  "/1
  Vsec/1 -> "PTS  "/1
  connections:
  "PTS  "/RConn1 -- "        "/RConn1
  "        "/RConn2 -- VRelay/LConn1
  Raux/LConn1 -- Rc+jXc/LConn1 -- "        "/LConn1 -- "CTS  "/RConn1
  Rc+jXc/RConn1 -- Raux/RConn1 -- "CTS  "/LConn1 -- "        "/LConn2
  VRelay/LConn2 -- "PTS  "/LConn1

== system IEEE13_coord/Regulator 1/Single Phase SVR_C/Transformer with Taps ==
  note: Vsec on Pt Ratio base
  note: Isec on CT Ratio base
  N : Inport
  "    " : Gain  Gain=1/ptRatio
  " 1" : Gain  Gain=1/ctRatio
  CT : spsCurrentMeasurementLib/Current Measurement  PhasorSimulation=off  OutputType=Complex  PSBequivalent=0
  Ground1 : spsGroundLib/Ground  LConnTagsString=a
  Ground2 : spsGroundLib/Ground  LConnTagsString=a
  Ground3 : spsGroundLib/Ground  LConnTagsString=a
  Memory : Memory
  Memory1 : Memory
  PT : spsVoltageMeasurementLib/Voltage Measurement  PhasorSimulation=off  OutputType=Complex  PSBequivalent=0
  "Variable-Ratio Transformer " : spsVariableRatioTransformerLib/Variable-Ratio Transformer
      settings: LibrarySourceBlock=|
      | sps_lib/Passives/Variable-Ratio
      | Transformer
  rs : spsSeriesRLCBranchLib/Series RLC Branch  LConnTagsString=__new0  RConnTagsString=__new0  BranchType=R  Resistance=1e-6  Inductance=1e-3  SetiL0=off  InitialCurrent=0  Capacitance=1e-6  Setx0=off  InitialVoltage=0  Measurements=None
  L : PMIOPort  Tag=PMCPort  Side=Right
  S : PMIOPort  Port=2  Side=Left
  Isec : Outport
  Vsec : Outport  Port=2
  wires:
  "    "/1 -> Memory1/1
  PT/1 -> "    "/1
  CT/1 -> " 1"/1
  " 1"/1 -> Memory/1
  N/1 -> "Variable-Ratio Transformer "/1
  Memory1/1 -> Vsec/1
  Memory/1 -> Isec/1
  connections:
  PT/LConn2 -- Ground1/LConn1
  rs/RConn1 -- CT/LConn1 -- PT/LConn1
  CT/RConn1 -- L/RConn1
  "Variable-Ratio Transformer "/RConn1 -- rs/LConn1
  Ground3/LConn1 -- "Variable-Ratio Transformer "/LConn2
  Ground2/LConn1 -- "Variable-Ratio Transformer "/RConn2
  S/RConn1 -- "Variable-Ratio Transformer "/LConn1

== system IEEE13_coord/Regulator 1/Single Phase SVR_C/Voltage Regulator Control ==
  note: N= 1/ (1+TapPosition*DeltaU)
  Vm : Inport
  1 : Constant
  Constant : Constant  Value=RegulatorOn
  Constant5 : Constant
  Product : Product  Inputs=/*
  Sum : Sum
  Tap Changer Control : Subsystem  mask(Tap Changer Control){MinMaxTap=TapMinMax, InitialPosition=InitialTap, MecDelay=TapSelectionTime}
      mask prompts: MinMaxTap "Minimum and maximum tap number [ Min  Max ] :"; InitialPosition "Initial tap position"; MecDelay "Mechanical delay time"
      mask init:
      | if MecDelay<=0,
      | 	MecDelay=1/60;
      | end
  Voltage change per tap : Gain  Gain=DeltaU
  Voltage regulator : Subsystem  mask{Vref=RegulatorVref*120, DeadBand=RegulatorDeadBand*120, TimeDelay=RegulatorDelay}
      mask prompts: Vref "Vref (on 120v base)"; DeadBand "Deadband (on 120v base)"; TimeDelay "Time delay (s)"
  N : Outport
  Tap : Outport  Port=2
  wires:
  Vm/1 -> Voltage regulator/1(Vmes (pu))
  Product/1 -> N/1
  Constant/1 -> Voltage regulator/3(RegOn)
  Tap Changer Control/2(Ready) -> Voltage regulator/2(Ready)
  Voltage change per tap/1 -> Sum/2
  Constant5/1 -> Sum/1
  Voltage regulator/1(Up) -> Tap Changer Control/1("Up ")
  Tap Changer Control/1(TapNo) -> Voltage change per tap/1, Tap/1  "Tap"
  1/1 -> Product/2
  Sum/1 -> Product/1
  Voltage regulator/2(Down) -> Tap Changer Control/2("Down ")

== system IEEE13_coord/Regulator 1/Single Phase SVR_A/Voltage Regulator Control/Tap Changer Control ==
  "Up " : Inport
  "Down " : Inport  Port=2
  Constant : Constant  Value=-1
  Constant1 : Constant
  Determine tap position : Subsystem
  Edge Detector : Subsystem  DialogController=POWERSYS.PowerSysDialog  mask(Edge Detector){model=Rising, ic=0}
      mask prompts: model "Edge:"; ic "Input at t = -eps:"
      mask help:
      | This block compares its present input to its previous input.
      |
      | If the input  is a logic signal (TRUE (1) or FALSE (0), the output is a one-step boolean signal TRUE  when  the specified edge (Rising, Falling or Either)  is detected.
      |
      | This block can also be used to detect the slope polarity of a continuous signal. For example, if the specified edge is  "Rising", the output is TRUE as long as the slope of the input signal is positive.
      |
      | The input value at time preceding t=0 is specified by the parameter "Input at t=-eps"
      mask init:
      | if model~=3,
      | 	x1 = (model -1)*20;
      |     x2 = (model -1)*60;
      | 	X1=[5,20,20,35]+25; Y1=[20+x2,20+x2,80-x2,80-x2];
      | 	X2=[5,20,35]+25;    Y2=[40+x1,60-x1,40+x1];
      | 	X3=[];X4=[];Y3=[];Y4=[];
      | else
      | 	x1 = 20;
      | 	x2 = 60;
      | 	X1=[5,20,20,35]+8; Y1=[20,20,80,80];
      | 	X2=[5,20,35]+8;    Y2=[40,60,40];
      | 	X3=[5,20,20,35]+53; Y3=[20+x2,20+x2,80-x2,80-x2];
      | 	X4=[5,20,35]+53;    Y4=[40+x1,60-x1,40+x1];
      | end
      | power_initmask();
      mask Help: This block is part of a subset of blocks in the Extras library that does not have documentation associated with it, other than the block mask description.
      mask TypeOptions model: Rising | Falling | Either
      mask Display: plot(0,0,100,100, X1,Y1,X2,Y2,X3,Y3,X4,Y4);
  Logical Operator : Logic  Operator=OR  AllPortsSameDT=off
  Logical Operator1 : Logic  AllPortsSameDT=off
  Mechanical Delay : TransportDelay  DelayTime=MecDelay  InitialOutput=InitialPosition  BufferSize=5120
  Memory : Memory  InitialCondition=1  InheritSampleTime=on
  Relational Operator : RelationalOperator  Operator===  OutDataTypeStr=float('double')  InputSameDT=off
  Switch : Switch  Threshold=0.5  InputSameDT=off
  TapNo : Outport  VectorParamsAs1DForOutWhenUnconnected=off
  Ready : Outport  Port=2  VectorParamsAs1DForOutWhenUnconnected=off
  wires:
  Edge Detector/1(Out) -> Logical Operator1/2
  Logical Operator/1 -> Edge Detector/1(In)
  Memory/1 -> Ready/1, Logical Operator1/1
  Relational Operator/1 -> Memory/1
  Determine tap position/1(TapNo) -> Relational Operator/1, Mechanical Delay/1
  Switch/1 -> Determine tap position/1(NewTap)
  Constant1/1 -> Switch/3
  Constant/1 -> Switch/1
  "Down "/1 -> Switch/2, Logical Operator/2
  "Up "/1 -> Logical Operator/1
  Logical Operator1/1 -> Determine tap position/Trigger
  Mechanical Delay/1 -> Relational Operator/2, TapNo/1

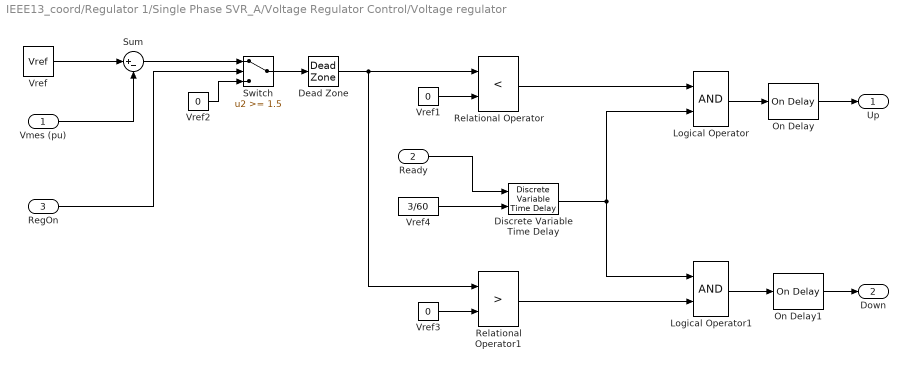
== system IEEE13_coord/Regulator 1/Single Phase SVR_A/Voltage Regulator Control/Voltage regulator ==
  Vmes (pu) : Inport
  Ready : Inport  Port=2
  RegOn : Inport  Port=3
  Dead Zone : DeadZone  LowerValue=-DeadBand/2  UpperValue=+DeadBand/2
  Discrete Variable Time Delay : spsDiscreteVariableTimeDelayLib/Discrete Variable Time Delay  MaxDelay=3/60+Ts  InitialValue=1  Ts=Ts  DFT=on
      settings: LibrarySourceBlock=|
      | sps_lib/Control/Discrete Variable
      | Time Delay
  Logical Operator : Logic  AllPortsSameDT=off
  Logical Operator1 : Logic  AllPortsSameDT=off
  On Delay : spsOnDelayLib/On Delay  DelayType=On delay  delay=TimeDelay  ic=0  Ts=Ts
  On Delay1 : spsOnDelayLib/On Delay  DelayType=On delay  delay=TimeDelay  ic=0  Ts=Ts
  Relational Operator : RelationalOperator  Operator=<  InputSameDT=off
  Relational Operator1 : RelationalOperator  Operator=>  InputSameDT=off
  Sum : Sum  Inputs=|+-  SaturateOnIntegerOverflow=on
  Switch : Switch  Threshold=1.5  InputSameDT=off
  Vref : Constant  Value=Vref
  Vref1 : Constant  Value=0
  Vref2 : Constant  Value=0
  Vref3 : Constant  Value=0
  Vref4 : Constant  Value=3/60
  Up : Outport  VectorParamsAs1DForOutWhenUnconnected=off
  Down : Outport  Port=2  VectorParamsAs1DForOutWhenUnconnected=off
  wires:
  Vref4/1 -> Discrete Variable Time Delay/2
  Discrete Variable Time Delay/1 -> Logical Operator/2, Logical Operator1/1
  Vref3/1 -> Relational Operator1/2
  On Delay1/1 -> Down/1
  Logical Operator1/1 -> On Delay1/1
  Relational Operator1/1 -> Logical Operator1/2
  On Delay/1 -> Up/1
  Logical Operator/1 -> On Delay/1
  Ready/1 -> Discrete Variable Time Delay/1
  Relational Operator/1 -> Logical Operator/1
  Vref1/1 -> Relational Operator/2
  Dead Zone/1 -> Relational Operator/1, Relational Operator1/1
  Vmes (pu)/1 -> Sum/2
  Vref/1 -> Sum/1
  Sum/1 -> Switch/1
  Switch/1 -> Dead Zone/1
  RegOn/1 -> Switch/2
  Vref2/1 -> Switch/3
